simulink model "energyAcct_Driveline"  (R2024a)
settings: Solver=VariableStepAuto  StartTime=0.0  StopTime=800  MaxStep=0.01  RelTol=1e-3  AbsTol=1e-3  EnableMultiTasking=on
PostLoadFcn:
  | energyAcct_Driveline_param
undefined symbols (not defined in the file or in its folder): drvEnAcc
libraries: sdl_lib x9, nesl_utility x8, fl_lib x8, simulink x5
Description:
  | Copyright 2023-2024 The MathWorks, Inc.
settings Model: Creator=smiller  LastModifiedBy=smiller
settings SolverCC: AutoScaleAbsTol=off  AlgebraicLoopSolver=TrustRegion  MaxZcPerStep=1
settings DataIOCC: LimitDataPoints=on  MaxDataPoints=10000  ReturnWorkspaceOutputs=off
settings OptimizationCC: ReuseModelBlockBuffer=off  LifeSpan=inf
settings DebuggingCC: UnconnectedInputMsg=warning  UnconnectedOutputMsg=warning  UnconnectedLineMsg=warning  AllowSymbolicDim=off  SubsystemReferenceDiagnosticForUnitTest=warning  SFUnexpectedBacktrackingDiag=warning  SFNoUnconditionalDefaultTransitionDiag=warning  SFExecutionAtInitializationDiag=none  ArithmeticOperatorsInVariantConditions=warning
settings ModelReferenceCC: EnableRefExpFcnMdlSchedulingChecks=on
settings SFSimCC: SimUseLocalCustomCode=off  CustomCodeUndefinedFunction=UseInterfaceOnly
settings RTWCC: RTWUseLocalCustomCode=off  GPUComputeCapability=3.5  DLArmComputeVersion=19.05
settings CodeAppCC: StateflowObjectComments=on
settings GRTTargetCC: TargetLangStandard=C89/C90 (ANSI)
settings ConfigComp: CovMetricSettings=dw  CovSaveCumulativeToWorkspaceVar=on  CovSaveSingleToWorkspaceVar=on  CovExternalEMLEnable=off  CovSFcnEnable=off
settings SimscapeCC: SimscapeLogType=all  SimscapeLogSimulationStatistics=on  SimscapeLogName=simlog_energyAcct_Driveline  SimscapeLogLimitData=off  SimscapeLogDataHistory=10000

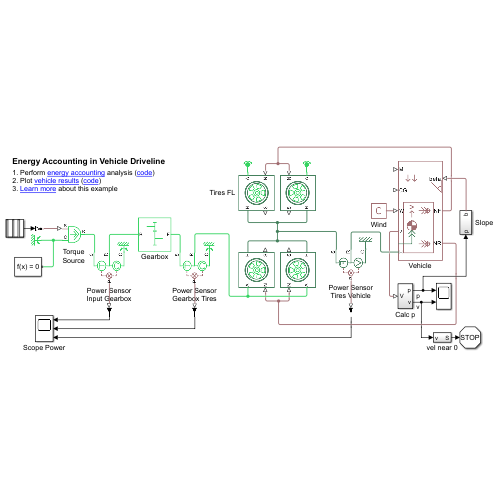
[thumbnail: Simulink's stored preview of the top-level diagram]
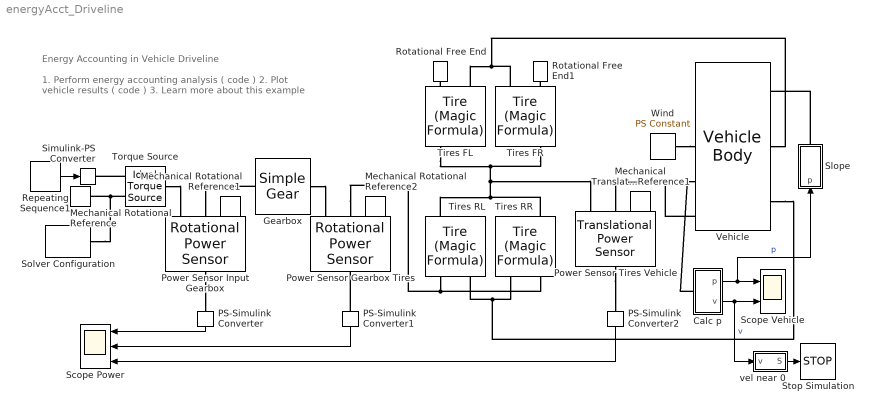
== system energyAcct_Driveline ==
  note: 1. Perform energy accounting analysis ( code )
      | 2. Plot vehicle results ( code )
      | 3. Learn more about this example
  note: Energy Accounting in Vehicle Driveline
  Calc p : Subsystem
  Gearbox : sdl_lib/Gears/Simple Gear  ratio=drvEnAcc.Gearbox.ratio  rotation_direction=sdl.enum.shaftOutputDirection.same  enable_faults=simscape.enum.onoff.off  efficiency_fault=0.05  fault_angles=pi / 12 rad  friction_model=sdl.enum.gear_efficiencies_load.constant  T_noload=0.1 N*m  T_nom=5 N*m  efficiency_nom=0.8  efficiency=drvEnAcc.Gearbox.eff  temperature_TLU=[280, 300, 320] K  load_TLU=[1, 5, 10] N*m  efficiency_TLU=[.95, .9, .85]  efficiency_TLU2=[.85, .8, .75; .95, .9, .85; .85, .8, .7]  w_thr=0.01 rad/s  pwr_thr=0.001 W  enable_backlash=false  hardstop_model=simscape.enum.hardstop.smooth  backlash_distance=1e-3 mm  r_base=0.1 m  transition=1e-4 mm  backlash_stiffness=1e6 N/m  backlash_damping=1e3 N*s/m  coeff_rest=0.7  v_tol=0.001 m/s  f_tol=0.001 N  mu_visc=drvEnAcc.Gearbox.visc N*m*s/rad  thermal_mass=50 J/K  temperature_specify=off  temperature_priority=High  temperature=300 K  temperature_nominal_specify=off  temperature_nominal_value=1  temperature_nominal_unit=K  x_backlash_specify=off  x_backlash_priority=None  x_backlash=0 mm  x_backlash_nominal_specify=off  x_backlash_nominal_value=1  x_backlash_nominal_unit=mm  f_hardstop_specify=off  f_hardstop_priority=None  f_hardstop=0 N  f_hardstop_nominal_specify=off  f_hardstop_nominal_value=1  f_hardstop_nominal_unit=N  v_backlash_specify=off  v_backlash_priority=None  v_backlash=0 m/s  v_backlash_nominal_specify=off  v_backlash_nominal_value=1  v_backlash_nominal_unit=m/s
  Mechanical Rotational Reference : fl_lib/Mechanical/Rotational Elements/Mechanical Rotational Reference
  Mechanical Rotational Reference1 : fl_lib/Mechanical/Rotational Elements/Mechanical Rotational Reference
  Mechanical Rotational Reference2 : fl_lib/Mechanical/Rotational Elements/Mechanical Rotational Reference
  Mechanical Translational Reference1 : fl_lib/Mechanical/Translational Elements/Mechanical Translational Reference
  PS-Simulink Converter : nesl_utility/PS-Simulink Converter  PhysicalDomain=network_engine_domain  SubClassName=ps_output  LeftPortType=input  RightPortType=output  PseudoPeriodic=off  Frequencies=[]  VectorFormat=inherit  Unit=inherit  AffineConversion=off
  PS-Simulink Converter1 : nesl_utility/PS-Simulink Converter  PhysicalDomain=network_engine_domain  SubClassName=ps_output  LeftPortType=input  RightPortType=output  PseudoPeriodic=off  Frequencies=[]  VectorFormat=inherit  Unit=inherit  AffineConversion=off
  PS-Simulink Converter2 : nesl_utility/PS-Simulink Converter  PhysicalDomain=network_engine_domain  SubClassName=ps_output  LeftPortType=input  RightPortType=output  PseudoPeriodic=off  Frequencies=[]  VectorFormat=inherit  Unit=inherit  AffineConversion=off
  Power Sensor Gearbox Tires : sdl_lib/Sensors/Rotational Power Sensor  measurement_type=sdl.enum.rotationalPowerSensorType.instantaneous  averaging_period=1 s  max_frequency=1000 Hz  max_speed=1000 rpm
      settings: InternalSimscapePortConfiguration="{\"Bottom\":[],\"Left\":[{\"id\":\"S\",\"label\":\"S\",\"type\":\"foundation.mechanical.rotational.rotational\"},{\"id\":\"R\",\"label\":\"R\",\"type\":\"foundation.mechanical.rotational.rotational\"},{\"id\":\"C\",\"label\":\"C\",\"type\":\"foundation.mechanical.rotational.rotational\"}],\"Right\":[{\"id\":\"P\",\"label\":\"P\",\"type\":\"output\"}],\"Top\":[]}"
  Power Sensor Input Gearbox : sdl_lib/Sensors/Rotational Power Sensor  measurement_type=sdl.enum.rotationalPowerSensorType.instantaneous  averaging_period=1 s  max_frequency=1000 Hz  max_speed=1000 rpm
      settings: InternalSimscapePortConfiguration="{\"Bottom\":[],\"Left\":[{\"id\":\"S\",\"label\":\"S\",\"type\":\"foundation.mechanical.rotational.rotational\"},{\"id\":\"R\",\"label\":\"R\",\"type\":\"foundation.mechanical.rotational.rotational\"},{\"id\":\"C\",\"label\":\"C\",\"type\":\"foundation.mechanical.rotational.rotational\"}],\"Right\":[{\"id\":\"P\",\"label\":\"P\",\"type\":\"output\"}],\"Top\":[]}"
  Power Sensor Tires Vehicle : sdl_lib/Sensors/Translational Power Sensor  measurement_type=sdl.enum.translationalPowerSensorType.instantaneous  averaging_period=1 s  max_frequency=1000 Hz
      settings: InternalSimscapePortConfiguration="{\"Bottom\":[],\"Left\":[{\"id\":\"S\",\"label\":\"S\",\"type\":\"foundation.mechanical.translational.translational\"},{\"id\":\"R\",\"label\":\"R\",\"type\":\"foundation.mechanical.translational.translational\"},{\"id\":\"C\",\"label\":\"C\",\"type\":\"foundation.mechanical.translational.translational\"}],\"Right\":[{\"id\":\"P\",\"label\":\"P\",\"type\":\"output\"}],\"Top\":[]}"
  Repeating Sequence1 : simulink/Sources/Repeating Sequence  rep_seq_t=[0 2 10 240 250 1000]  rep_seq_y=[0 0 500 500 0 0]*drvEnAcc.Scenario.trqscale
  Rotational Free End : fl_lib/Mechanical/Rotational Elements/Rotational Free End  w_specify=off  w_priority=None  w=0 rad/s  w_nominal_specify=off  w_nominal_value=1  w_nominal_unit=rad/s
  Rotational Free End1 : fl_lib/Mechanical/Rotational Elements/Rotational Free End  w_specify=off  w_priority=None  w=0 rad/s  w_nominal_specify=off  w_nominal_value=1  w_nominal_unit=rad/s
  Scope Vehicle : Scope  NumInputPorts=2
  Scope Power : Scope  NumInputPorts=3
  Simulink-PS Converter : nesl_utility/Simulink-PS Converter  PhysicalDomain=network_engine_domain  SubClassName=ps_input  LeftPortType=input  RightPortType=output  PseudoPeriodic=off  Frequencies=[]  NoiseDistribution=none  NoiseParameters=[]  Unit=1  AffineConversion=off  FilteringAndDerivatives=filter  SimscapeFilterOrder=1  InputFilterTimeConstant=0.01  UdotUserProvided=0
  Slope : Subsystem
  Solver Configuration : nesl_utility/Solver Configuration  PhysicalDomain=network_engine_domain  SubClassName=solver  LeftPortType=input  RightPortType=generic  Tones=[]  Harmonics=[]  SimulateNoise=off  Profile=off  UseLocalSampling=off  EnableSwitchedLinearOptims=on  FrequencyDomain=off  UseCCode=off  RelTol=0.001  AbsTol=1e-06  MinStep=1e-09  ToWorkspace=off  RevertToSquareIcSolve=off  NumHomotopyIterations=100  PhasorMode=off  PhasorModeNumHarmonics=1  ConsistencySolver=NEWTON_XTOL_AFTER_FTOL  IndexReductionMethod=DerivativeReplacement  DoDC=off  ResidualTolerance=1e-09  ConsistencyTolSource=GLOBAL  ConsistencyAbsTol=0.001  ConsistencyRelTol=0.001  ConsistencyTolFactor=0.001  UseLocalSolver=off  LocalSolverChoice=NE_BACKWARD_EULER_ADVANCER  ResolveIndetEquations=on  FunctionEvalNumThread=1  LocalSolverSampleTime=0.1  DoFixedCost=off  MaxNonlinIter=3  MaxModeIter=2  ComputeImpulses=off  ImpulseIterations=2  LinearAlgebra=auto  LinearAlgebraNumThread=0  EquationFormulation=NE_TIME_EF  DelaysMemoryBudget=1024  AutomaticFiltering=on  FilteringTimeConstant=0.001  PartitionStorageMethod=AS_NEEDED  PartitionMemoryBudget=1024  PartitionMethod=ROBUST  MultibodyUseLocalSolver=off  MultibodyLocalSolverChoice=ODE1  MultibodyLocalSolverSampleTime=0.001
  Stop Simulation : Stop
  Tires FL : sdl_lib/Tires & Vehicles/Tire (Magic Formula)  parameterization=sdl.enum.magic_tire_model.peak  F_z1=3000 N  F_x1=3500 N  kappa1=10  B_m=10  C_m=1.9  D_m=1  E_m=0.97  fz0=4000 N  p_Cx=1.685  p_Dx=[1.21, -.037]  p_Ex=[.344, .095, -.02, 0]  p_Kx=[21.51, -.163, .245]  p_Hx=[-.002, .002]  p_Vx=[0, 0]  rolling_radius_model=sdl.enum.RollingRadiusParameterization.Constant  r_e=drvEnAcc.Tire.radius m  r_0=0.3 m  breff=8.39  dreff=0.26  freff=0.074  q_re0=0.99  q_v1=0.008  longvl=17 m/s  cz=5e5 N/m  model_resistance=true  resistance_model=sdl.enum.rollingResistanceParameterization.constant  coeff=drvEnAcc.Tire.resist.coeff  p_tire=250e3 Pa  alpha=-0.003  beta=0.97  coeff_a=84e-4  coeff_b=6.2e-4 s/m  coeff_c=1.6e-4 s^2/m^2  p_tire0=240e3 Pa  fz0_resistance=4000 N  vH0=16 m/s  q_Sy=[.0082, 0, .0014, .001, 0, 0, 1.08, -.5]  v_thr=drvEnAcc.Tire.resist.thresh m/s  enable_scaling_coefficients=false  lfzO=1  lcx=1  lmux=1  lex=1  lkx=1  lhx=1  lvx=1  lmy=1  model_compliance=sdl.enum.compliance.off  stiffness=1e6 N/m  damping=1000 N*s/m  model_inertia=sdl.enum.model_inertia.on  inertia=drvEnAcc.Tire.inertia kg*m^2  initial_velocity=0 rad/s  vxlow=1 m/s  v_tr_thr=0.1 m/s  kpumin=-1.5  kpumax=1.5
  Tires FR : sdl_lib/Tires & Vehicles/Tire (Magic Formula)  parameterization=sdl.enum.magic_tire_model.peak  F_z1=3000 N  F_x1=3500 N  kappa1=10  B_m=10  C_m=1.9  D_m=1  E_m=0.97  fz0=4000 N  p_Cx=1.685  p_Dx=[1.21, -.037]  p_Ex=[.344, .095, -.02, 0]  p_Kx=[21.51, -.163, .245]  p_Hx=[-.002, .002]  p_Vx=[0, 0]  rolling_radius_model=sdl.enum.RollingRadiusParameterization.Constant  r_e=drvEnAcc.Tire.radius m  r_0=0.3 m  breff=8.39  dreff=0.26  freff=0.074  q_re0=0.99  q_v1=0.008  longvl=17 m/s  cz=5e5 N/m  model_resistance=true  resistance_model=sdl.enum.rollingResistanceParameterization.constant  coeff=drvEnAcc.Tire.resist.coeff  p_tire=250e3 Pa  alpha=-0.003  beta=0.97  coeff_a=84e-4  coeff_b=6.2e-4 s/m  coeff_c=1.6e-4 s^2/m^2  p_tire0=240e3 Pa  fz0_resistance=4000 N  vH0=16 m/s  q_Sy=[.0082, 0, .0014, .001, 0, 0, 1.08, -.5]  v_thr=drvEnAcc.Tire.resist.thresh m/s  enable_scaling_coefficients=false  lfzO=1  lcx=1  lmux=1  lex=1  lkx=1  lhx=1  lvx=1  lmy=1  model_compliance=sdl.enum.compliance.off  stiffness=1e6 N/m  damping=1000 N*s/m  model_inertia=sdl.enum.model_inertia.on  inertia=drvEnAcc.Tire.inertia kg*m^2  initial_velocity=0 rad/s  vxlow=1 m/s  v_tr_thr=0.1 m/s  kpumin=-1.5  kpumax=1.5
  Tires RL : sdl_lib/Tires & Vehicles/Tire (Magic Formula)  parameterization=sdl.enum.magic_tire_model.peak  F_z1=3000 N  F_x1=3500 N  kappa1=10  B_m=10  C_m=1.9  D_m=1  E_m=0.97  fz0=4000 N  p_Cx=1.685  p_Dx=[1.21, -.037]  p_Ex=[.344, .095, -.02, 0]  p_Kx=[21.51, -.163, .245]  p_Hx=[-.002, .002]  p_Vx=[0, 0]  rolling_radius_model=sdl.enum.RollingRadiusParameterization.Constant  r_e=drvEnAcc.Tire.radius m  r_0=0.3 m  breff=8.39  dreff=0.26  freff=0.074  q_re0=0.99  q_v1=0.008  longvl=17 m/s  cz=5e5 N/m  model_resistance=true  resistance_model=sdl.enum.rollingResistanceParameterization.constant  coeff=drvEnAcc.Tire.resist.coeff  p_tire=250e3 Pa  alpha=-0.003  beta=0.97  coeff_a=84e-4  coeff_b=6.2e-4 s/m  coeff_c=1.6e-4 s^2/m^2  p_tire0=240e3 Pa  fz0_resistance=4000 N  vH0=16 m/s  q_Sy=[.0082, 0, .0014, .001, 0, 0, 1.08, -.5]  v_thr=drvEnAcc.Tire.resist.thresh m/s  enable_scaling_coefficients=false  lfzO=1  lcx=1  lmux=1  lex=1  lkx=1  lhx=1  lvx=1  lmy=1  model_compliance=sdl.enum.compliance.off  stiffness=1e6 N/m  damping=1000 N*s/m  model_inertia=sdl.enum.model_inertia.on  inertia=drvEnAcc.Tire.inertia kg*m^2  initial_velocity=0 rad/s  vxlow=1 m/s  v_tr_thr=0.1 m/s  kpumin=-1.5  kpumax=1.5
  Tires RR : sdl_lib/Tires & Vehicles/Tire (Magic Formula)  parameterization=sdl.enum.magic_tire_model.peak  F_z1=3000 N  F_x1=3500 N  kappa1=10  B_m=10  C_m=1.9  D_m=1  E_m=0.97  fz0=4000 N  p_Cx=1.685  p_Dx=[1.21, -.037]  p_Ex=[.344, .095, -.02, 0]  p_Kx=[21.51, -.163, .245]  p_Hx=[-.002, .002]  p_Vx=[0, 0]  rolling_radius_model=sdl.enum.RollingRadiusParameterization.Constant  r_e=drvEnAcc.Tire.radius m  r_0=0.3 m  breff=8.39  dreff=0.26  freff=0.074  q_re0=0.99  q_v1=0.008  longvl=17 m/s  cz=5e5 N/m  model_resistance=true  resistance_model=sdl.enum.rollingResistanceParameterization.constant  coeff=drvEnAcc.Tire.resist.coeff  p_tire=250e3 Pa  alpha=-0.003  beta=0.97  coeff_a=84e-4  coeff_b=6.2e-4 s/m  coeff_c=1.6e-4 s^2/m^2  p_tire0=240e3 Pa  fz0_resistance=4000 N  vH0=16 m/s  q_Sy=[.0082, 0, .0014, .001, 0, 0, 1.08, -.5]  v_thr=drvEnAcc.Tire.resist.thresh m/s  enable_scaling_coefficients=false  lfzO=1  lcx=1  lmux=1  lex=1  lkx=1  lhx=1  lvx=1  lmy=1  model_compliance=sdl.enum.compliance.off  stiffness=1e6 N/m  damping=1000 N*s/m  model_inertia=sdl.enum.model_inertia.on  inertia=drvEnAcc.Tire.inertia kg*m^2  initial_velocity=0 rad/s  vxlow=1 m/s  v_tr_thr=0.1 m/s  kpumin=-1.5  kpumax=1.5
  Torque Source : fl_lib/Mechanical/Mechanical Sources/Ideal Torque Source
  Vehicle : sdl_lib/Tires & Vehicles/Vehicle Body  mass=drvEnAcc.Vehicle.mass kg  n_w=2  x_f=drvEnAcc.Vehicle.CG2FA m  x_r=drvEnAcc.Vehicle.CG2RA m  y_c=drvEnAcc.Vehicle.CG2gnd m  mass_var=simscape.enum.onoff.on  g=9.81 m/s^2  liftoff_warning=simscape.enum.onoff.on  area=drvEnAcc.Vehicle.areaF m^2  Cd=drvEnAcc.Vehicle.cD  rho=drvEnAcc.Vehicle.rhoAir kg/m^3  model_pitch=simscape.enum.onoff.off  inertia=4000 kg*m^2  suspension_model=sdl.enum.linearTLU.linear  k_f=1e4 N/m  b_f=1e4 N*s/m  k_r=1e4 N/m  b_r=1e4 N*s/m  k_f_TLU=[-2000, -1000, 0, 1000, 2000] N  x_f_TLU=[-.4, -.2, 0, .2, .4] m  b_f_TLU=[-200, -100, 0, 100, 200] N  v_f_TLU=[-4, -2, 0, 2, 4] m/s  k_r_TLU=[-2000, -1000, 0, 1000, 2000] N  x_r_TLU=[-.4, -.2, 0, .2, .4] m  b_r_TLU=[-200, -100, 0, 100, 200] N  v_r_TLU=[-4, -2, 0, 2, 4] m/s  interp_method=simscape.enum.interpolation.linear  extrap_method=simscape.enum.extrapolation.linear  model_hardstop=simscape.enum.onoff.off  upper_bound_f=.25 m  lower_bound_f=-.25 m  stop_k_f=1e6 N/m  stop_b_f=150 N*s/m  upper_bound_r=.25 m  lower_bound_r=-.25 m  stop_k_r=1e6 N/m  stop_b_r=150 N*s/m  initial_pitch=0 rad  initial_pitch_rate=0 rad/s  v_specify=on  v_priority=High  v=0 m/s  v_nominal_specify=off  v_nominal_value=1  v_nominal_unit=m/s
      settings: InternalSimscapePortConfiguration="{\"Bottom\":[],\"Left\":[{\"id\":\"H\",\"label\":\"H\",\"type\":\"foundation.mechanical.translational.translational\"},{\"id\":\"V\",\"label\":\"V\",\"type\":\"output\"},{\"id\":\"wind\",\"label\":\"W\",\"type\":\"input\"},{\"id\":\"cg_load\",\"label\":\"CG\",\"type\":\"input\"},{\"id\":\"mass_load\",\"label\":\"M\",\"type\":\"input\"}],\"Right\":[{\"id\":\"NR\",\"label\":\"NR\",\"type\":\"output\"},{\"id\":\"NF\",\"label\":\"NF\",\"type\":\"output\"},{\"id\":\"beta\",\"label\":\"beta\",\"type\":\"input\"}],\"Top\":[]}"
  Wind : fl_lib/Physical Signals/Sources/PS Constant  constant=drvEnAcc.Scenario.wind m/s
  vel near 0 : Subsystem
  wires:
  Repeating Sequence1/1 -> Simulink-PS Converter/1
  PS-Simulink Converter/1 -> Scope Power/1
  PS-Simulink Converter1/1 -> Scope Power/2
  Calc p/1(p) -> Slope/1(p), Scope Vehicle/1  "p"
  Calc p/2(v) -> Scope Vehicle/2, vel near 0/1(v)  "v"
  PS-Simulink Converter2/1 -> Scope Power/3
  vel near 0/1(S) -> Stop Simulation/1
  connections:
  Power Sensor Gearbox Tires/LConn2 -- Tires RR/LConn2 -- Tires RL/LConn2
  Torque Source/LConn1 -- Power Sensor Input Gearbox/LConn1
  Solver Configuration/RConn1 -- Torque Source/RConn2 -- Mechanical Rotational Reference/LConn1
  Torque Source/RConn1 -- Simulink-PS Converter/RConn1
  Power Sensor Input Gearbox/LConn3 -- Mechanical Rotational Reference1/LConn1
  Gearbox/LConn1 -- Power Sensor Input Gearbox/LConn2
  Power Sensor Input Gearbox/RConn1 -- PS-Simulink Converter/LConn1
  Gearbox/RConn1 -- Power Sensor Gearbox Tires/LConn1
  Mechanical Rotational Reference2/LConn1 -- Power Sensor Gearbox Tires/LConn3
  PS-Simulink Converter1/LConn1 -- Power Sensor Gearbox Tires/RConn1
  Power Sensor Tires Vehicle/LConn1 -- Tires RR/RConn2 -- Tires RL/RConn2 -- Tires FR/RConn2 -- Tires FL/RConn2
  Vehicle/RConn2 -- Tires FR/LConn1 -- Tires FL/LConn1
  Vehicle/RConn1 -- Tires RR/LConn1 -- Tires RL/LConn1
  Tires FR/LConn2 -- Rotational Free End1/LConn1
  Wind/RConn1 -- Vehicle/LConn3
  Tires FL/LConn2 -- Rotational Free End/LConn1
  Slope/RConn1 -- Vehicle/RConn3
  Vehicle/LConn1 -- Power Sensor Tires Vehicle/LConn2
  Power Sensor Tires Vehicle/LConn3 -- Mechanical Translational Reference1/LConn1
  Power Sensor Tires Vehicle/RConn1 -- PS-Simulink Converter2/LConn1
  Calc p/LConn1 -- Vehicle/LConn2

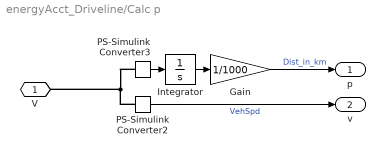
== system energyAcct_Driveline/Calc p ==
  Gain : Gain  Gain=1/1000
  Integrator : Integrator
  PS-Simulink Converter2 : nesl_utility/PS-Simulink Converter  PhysicalDomain=network_engine_domain  SubClassName=ps_output  LeftPortType=input  RightPortType=output  PseudoPeriodic=off  Frequencies=[]  VectorFormat=inherit  Unit=km/hr  AffineConversion=off
  PS-Simulink Converter3 : nesl_utility/PS-Simulink Converter  PhysicalDomain=network_engine_domain  SubClassName=ps_output  LeftPortType=input  RightPortType=output  PseudoPeriodic=off  Frequencies=[]  VectorFormat=inherit  Unit=m/s  AffineConversion=off
  V : PMIOPort  Side=Left
  p : Outport
  v : Outport  Port=2
  wires:
  PS-Simulink Converter3/1 -> Integrator/1
  Integrator/1 -> Gain/1
  PS-Simulink Converter2/1 -> v/1  "VehSpd"
  Gain/1 -> p/1  "Dist_in_km"
  connections:
  PS-Simulink Converter3/LConn1 -- PS-Simulink Converter2/LConn1 -- V/RConn1

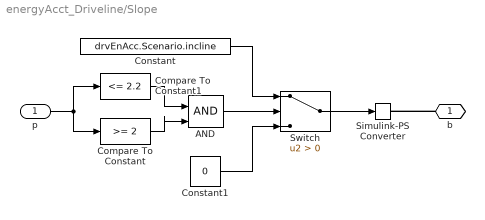
== system energyAcct_Driveline/Slope ==
  p : Inport
  AND : Logic  IconShape=distinctive  AllPortsSameDT=off  OutDataTypeStr=boolean
  Compare To Constant : simulink/Logic and Bit Operations/Compare To Constant  relop=>=  const=2  OutDataTypeStr=boolean  ZeroCross=off
  Compare To Constant1 : simulink/Logic and Bit Operations/Compare To Constant  relop=<=  const=2.2  OutDataTypeStr=boolean  ZeroCross=off
  Constant : Constant  Value=drvEnAcc.Scenario.incline
  Constant1 : Constant  Value=0
  Simulink-PS Converter : nesl_utility/Simulink-PS Converter  PhysicalDomain=network_engine_domain  SubClassName=ps_input  LeftPortType=input  RightPortType=output  PseudoPeriodic=off  Frequencies=[]  NoiseDistribution=none  NoiseParameters=[]  Unit=deg  AffineConversion=off  FilteringAndDerivatives=filter  SimscapeFilterOrder=1  InputFilterTimeConstant=0.1  UdotUserProvided=0
  Switch : Switch  Criteria=u2 > Threshold  SaturateOnIntegerOverflow=off  InputSameDT=off
  b : PMIOPort  Side=Right
  wires:
  Compare To Constant/1 -> AND/2
  p/1 -> Compare To Constant/1, Compare To Constant1/1
  Switch/1 -> Simulink-PS Converter/1
  Compare To Constant1/1 -> AND/1
  AND/1 -> Switch/2
  Constant/1 -> Switch/1
  Constant1/1 -> Switch/3
  connections:
  b/RConn1 -- Simulink-PS Converter/RConn1

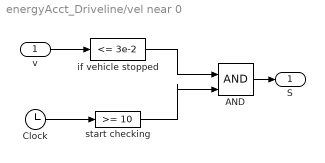
== system energyAcct_Driveline/vel near 0 ==
  v : Inport
  AND : Logic  IconShape=distinctive  AllPortsSameDT=off  OutDataTypeStr=boolean
  Clock : Clock
  if vehicle stopped : simulink/Logic and Bit Operations/Compare To Constant  relop=<=  const=3e-2  OutDataTypeStr=boolean
  start checking : simulink/Logic and Bit Operations/Compare To Constant  relop=>=  const=10  OutDataTypeStr=boolean
  S : Outport
  wires:
  start checking/1 -> AND/2
  AND/1 -> S/1
  if vehicle stopped/1 -> AND/1
  Clock/1 -> start checking/1
  v/1 -> if vehicle stopped/1
